simulink model "hysteretic_buck"  (R2025b)
settings: Solver=ode23tb  StartTime=0.0  StopTime=5e-3  MaxStep=1e-6  RelTol=1e-3
values from neighbouring files (symbols this model uses):
  C = 500e-6    (= 0.0005)    [buck_converter_parameters_A01.m]    (also in hysteretic_control_Buck_converter_V01.m = 0.0001; hysteretic_controller_simu_A01.m = 0.0001; type_1_compansator_A01.m = 1e-05)
  Ki = 100    [buck_converter_parameters_A01.m]    (also in hysteretic_controller_simu_A01.m = 1000)
  Kp = 80    [buck_converter_parameters_A01.m]    (also in hysteretic_controller_simu_A01.m = 1)
  L = 50e-6    (= 5e-05)    [buck_converter_parameters_A01.m]    (also in hysteretic_control_Buck_converter_V01.m = 0.0001; hysteretic_controller_simu_A01.m = 0.0001)
  R = 3    [buck_converter_parameters_A01.m]    (also in hysteretic_control_Buck_converter_V01.m; hysteretic_controller_simu_A01.m = 5; type_1_compansator_A01.m = 15.9154943092)
  Rs = 1    [hysteretic_controller_simu_A01.m]
  Vhys = 0.01    [buck_converter_parameters_A01.m]    (also in hysteretic_controller_simu_A01.m = 0.2; latched_hysteretic_circuit_A01.m = 0.5)
  Vin = 12    [hysteretic_controller_simu_A01.m]
settings Model: Creator=arif  LastModifiedBy=arif

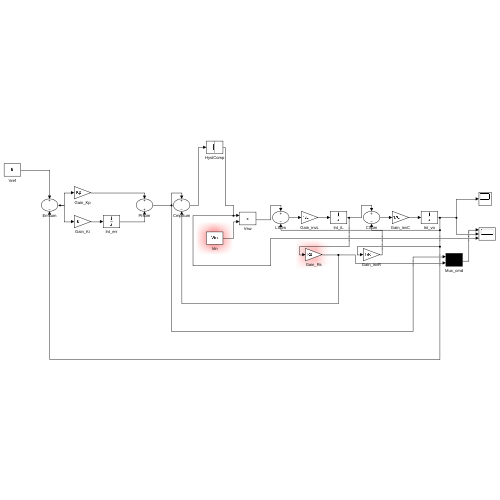
[thumbnail: Simulink's stored preview of the top-level diagram]
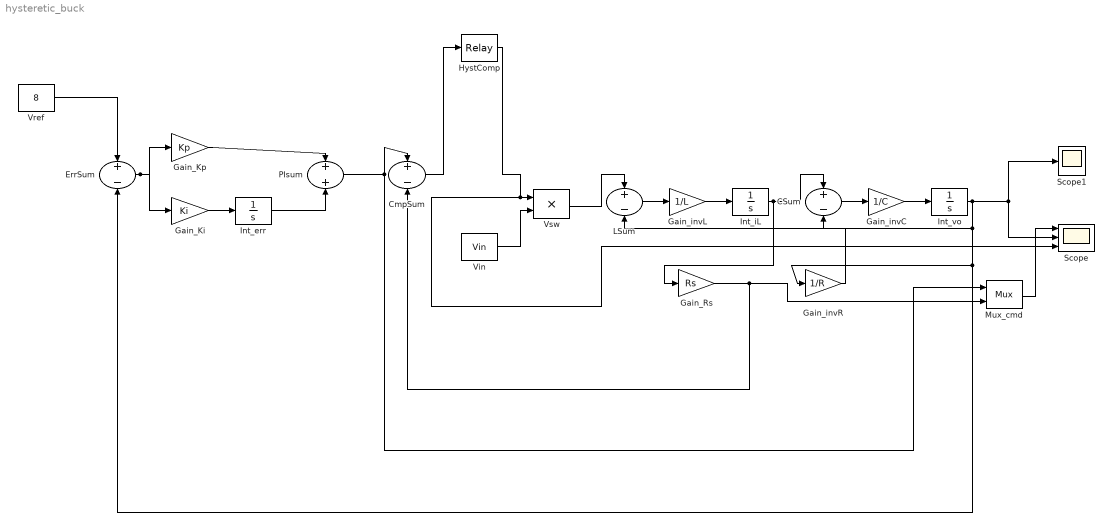
== system hysteretic_buck ==
  CSum : Sum  Inputs=+-
  CmpSum : Sum  Inputs=+-
  ErrSum : Sum  Inputs=+-
  Gain_Ki : Gain  Gain=Ki
  Gain_Kp : Gain  Gain=Kp
  Gain_Rs : Gain  Gain=Rs
  Gain_invC : Gain  Gain=1/C
  Gain_invL : Gain  Gain=1/L
  Gain_invR : Gain  Gain=1/R
  HystComp : Relay  OnSwitchValue=Vhys/2  OffSwitchValue=-Vhys/2
  Int_err : Integrator
  Int_iL : Integrator
  Int_vo : Integrator
  LSum : Sum  Inputs=+-
  Mux_cmd : Mux  Inputs=2
  PIsum : Sum
  Scope : Scope  NumInputPorts=3
      settings: ActiveDisplayYMinimum=-1  ActiveDisplayYMaximum=1
  Scope1 : Scope
      settings: ActiveDisplayYMinimum=-0.99916724363121434  ActiveDisplayYMaximum=8.99250519268093
  Vin : Constant  Value=Vin
  Vref : Constant  Value=8
  Vsw : Product
  wires:
  Vref/1 -> ErrSum/1
  Int_vo/1 -> ErrSum/2, Gain_invR/1, LSum/2, Scope/2, Scope1/1
  ErrSum/1 -> Gain_Kp/1, Gain_Ki/1
  Gain_Ki/1 -> Int_err/1
  Gain_Kp/1 -> PIsum/1
  Int_err/1 -> PIsum/2
  PIsum/1 -> CmpSum/1, Mux_cmd/1
  Gain_Rs/1 -> CmpSum/2, Mux_cmd/2
  CmpSum/1 -> HystComp/1
  HystComp/1 -> Vsw/1, Scope/3
  Vin/1 -> Vsw/2
  Vsw/1 -> LSum/1
  LSum/1 -> Gain_invL/1
  Gain_invL/1 -> Int_iL/1
  Int_iL/1 -> CSum/1, Gain_Rs/1
  Gain_invR/1 -> CSum/2
  CSum/1 -> Gain_invC/1
  Gain_invC/1 -> Int_vo/1
  Mux_cmd/1 -> Scope/1
